simulink model "VoltageSourceConverterHVDCTrans"  (R2025b)
settings: Solver=FixedStepDiscrete  StartTime=0.0  StopTime=5  FixedStep=Ts  MaxStep=1e-4  RelTol=1e-3
PreLoadFcn:
  | VoltageSourceConverterHVDCTransParameters
values from neighbouring files (symbols this model uses):
  c = 0.207e-6    (= 2.07e-07)    [VoltageSourceConverterHVDCTransParameters.m]
  Cf = ((QRatedFilter/(VRated^2*(2*pi*FRated)))*(n^2-1)/(n^2))/Cbase    [VoltageSourceConverterHVDCTransParameters.m]
  FRated = 60    [VoltageSourceConverterHVDCTransParameters.m]
  Idcbase = Pbase/VdcRated    (= 1000)    [VoltageSourceConverterHVDCTransParameters.m]
  IL0 = opIdc.get("I").Value.value    [VoltageSourceConverterHVDCTransInitializeModel.m]
  l = 0.189e-3    (= 0.000189)    [VoltageSourceConverterHVDCTransParameters.m]
  Lbase = Zbase/wbase    [VoltageSourceConverterHVDCTransParameters.m]
  Lr = 0.15    [VoltageSourceConverterHVDCTransParameters.m]
  n = 25    [VoltageSourceConverterHVDCTransParameters.m]
  PRated = 300e6    (= 300000000)    [VoltageSourceConverterHVDCTransParameters.m]
  r = 0.0376    [VoltageSourceConverterHVDCTransParameters.m]
  Rc = r*Dis    (= 11.28)    [VoltageSourceConverterHVDCTransParameters.m]
  Rr = 0.002    [VoltageSourceConverterHVDCTransParameters.m]
  Rt = 0.002625    [VoltageSourceConverterHVDCTransParameters.m]
  Ts = 1/(fsw*100)    [VoltageSourceConverterHVDCTransInitializeModel.m]    (also in VoltageSourceConverterHVDCTransParameters.m = 6.66666666667e-05; VoltageSourceConverterHVDCTransVariantControl.m)
  Tsc = 10*Ts    (= 0.166666666667)    [VoltageSourceConverterHVDCTransInitializeModel.m]    (also in VoltageSourceConverterHVDCTransParameters.m = 6.66666666667e-05; VoltageSourceConverterHVDCTransVariantControl.m)
  Vdcr0 = 2*opReceivingEndVdcp.get("V").Value.value    [VoltageSourceConverterHVDCTransInitializeModel.m]
  VdcRated = 300e3    (= 300000)    [VoltageSourceConverterHVDCTransParameters.m]
  Vdcs0 = 2*opSendingEndVdcp.get("V").Value.value    [VoltageSourceConverterHVDCTransInitializeModel.m]
  VRated = 150e3    (= 150000)    [VoltageSourceConverterHVDCTransParameters.m]
  Xt = 0.19197    [VoltageSourceConverterHVDCTransParameters.m]
  Zbase = Vbase/Ibase    [VoltageSourceConverterHVDCTransParameters.m]
undefined symbols (not defined in the file or in its folder): DiscIntNeverNeededParam
libraries: nesl_utility x43, fl_lib x32, ee_lib x22, eeTransforms x16, eeGeneralControl x14, slpidlib x13, mcbeeMathTransformLib x8, eeSinusoidalMeasurement x2, eePwmGeneratorThreeLevel x2
(part 2 of 4)

== system VoltageSourceConverterHVDCTrans/Sending end DC filter ==
  Bus Creator : BusCreator  Inputs=4
  Cfns : fl_lib/Electrical/Electrical Elements/Capacitor  c=Cdcf F  r=0 Ohm  g=0 1/Ohm  i_specify=off  i_priority=High  i=0 A  i_nominal_specify=off  i_nominal_value=1  i_nominal_unit=A  v_specify=off  v_priority=High  v=Vdcs0/2 V  v_nominal_specify=off  v_nominal_value=1  v_nominal_unit=V  vc_specify=on  vc_priority=High  vc=Vdcs0/2 V  vc_nominal_specify=off  vc_nominal_value=1  vc_nominal_unit=V
  Cfps : fl_lib/Electrical/Electrical Elements/Capacitor  c=Cdcf F  r=0 Ohm  g=0 1/Ohm  i_specify=off  i_priority=High  i=0 A  i_nominal_specify=off  i_nominal_value=1  i_nominal_unit=A  v_specify=off  v_priority=High  v=Vdcs0/2 V  v_nominal_specify=off  v_nominal_value=1  v_nominal_unit=V  vc_specify=on  vc_priority=High  vc=Vdcs0/2 V  vc_nominal_specify=off  vc_nominal_value=1  vc_nominal_unit=V
  Cns : fl_lib/Electrical/Electrical Elements/Capacitor  c=Cdc F  r=1e-3 Ohm  g=0 1/Ohm  i_specify=off  i_priority=High  i=0 A  i_nominal_specify=off  i_nominal_value=1  i_nominal_unit=A  v_specify=off  v_priority=High  v=Vdcs0/2 V  v_nominal_specify=off  v_nominal_value=1  v_nominal_unit=V  vc_specify=on  vc_priority=High  vc=Vdcs0/2 V  vc_nominal_specify=off  vc_nominal_value=1  vc_nominal_unit=V
  Cps : fl_lib/Electrical/Electrical Elements/Capacitor  c=Cdc F  r=1e-3 Ohm  g=0 1/Ohm  i_specify=off  i_priority=High  i=0 A  i_nominal_specify=off  i_nominal_value=1  i_nominal_unit=A  v_specify=off  v_priority=High  v=Vdcs0/2 V  v_nominal_specify=off  v_nominal_value=1  v_nominal_unit=V  vc_specify=on  vc_priority=High  vc=Vdcs0/2 V  vc_nominal_specify=off  vc_nominal_value=1  vc_nominal_unit=V
  Electrical Reference : fl_lib/Electrical/Electrical Elements/Electrical Reference
  Lfns : fl_lib/Electrical/Electrical Elements/Inductor  l=L2 H  r=0.05 Ohm  g=0 1/Ohm  i_specify=off  i_priority=None  i=0 A  i_nominal_specify=off  i_nominal_value=1  i_nominal_unit=A  v_specify=off  v_priority=None  v=0 V  v_nominal_specify=off  v_nominal_value=1  v_nominal_unit=V  i_L_specify=on  i_L_priority=High  i_L=-IL0 A  i_L_nominal_specify=off  i_L_nominal_value=1  i_L_nominal_unit=A
  Lfps : fl_lib/Electrical/Electrical Elements/Inductor  l=L2 H  r=0.05 Ohm  g=0 1/Ohm  i_specify=off  i_priority=High  i=0 A  i_nominal_specify=off  i_nominal_value=1  i_nominal_unit=A  v_specify=off  v_priority=None  v=0 V  v_nominal_specify=off  v_nominal_value=1  v_nominal_unit=V  i_L_specify=on  i_L_priority=High  i_L=IL0 A  i_L_nominal_specify=off  i_L_nominal_value=1  i_L_nominal_unit=A
  Lfs : fl_lib/Electrical/Electrical Elements/Inductor  l=L1 H  r=0.1 Ohm  g=0 1/Ohm  i_specify=off  i_priority=None  i=0 A  i_nominal_specify=off  i_nominal_value=1  i_nominal_unit=A  v_specify=off  v_priority=None  v=0 V  v_nominal_specify=off  v_nominal_value=1  v_nominal_unit=V  i_L_specify=on  i_L_priority=None  i_L=0 A  i_L_nominal_specify=off  i_L_nominal_value=1  i_L_nominal_unit=A
  Sensing current1 : Subsystem
      settings: PortSchema="{\"entries\":[{\"content\":{\"sides\":[{\"content\":{\"connectorIds\":[\"LConn1\"]},\"type\":\"ConnectorPlacement.EquallySpacedRectSide\",\"uuid\":\"b182dbc5-c8d5-4832-a7cd-ea3787954646\"},{\"content\":{\"connectorIds\":[\"RConn1\",\"Out1\"],\"side\":\"RIGHT\"},\"type\":\"ConnectorPlacement.EquallySpacedRectSide\",\"uuid\":\"bfc6f163-1abf-440b-aa89-1443f971fd07\"},{\"content\":{\"connectorIds\":[],\"side\":\"TOP\"},\"type\":\"ConnectorPlacement.EquallySpacedRectSide\",\"uuid\":\"dd2a104c-9a72-483e-91c4-dbef9b359450\"}]},\"type\":\"ConnectorPlacement.EquallySpacedConnector\",\"uuid\":\"ce98cc3b-f524-409d-a465-fff2e3b7df79\"}],\"packageUris\":[\"http://schema.mathworks.com/mf0/Connector/R2020b\"],\"version\":\"1.0\"}"
  Sensing current2 : Subsystem
      settings: PortSchema="{\"entries\":[{\"content\":{\"sides\":[{\"content\":{\"connectorIds\":[\"LConn1\"]},\"type\":\"ConnectorPlacement.EquallySpacedRectSide\",\"uuid\":\"b182dbc5-c8d5-4832-a7cd-ea3787954646\"},{\"content\":{\"connectorIds\":[\"RConn1\",\"Out1\"],\"side\":\"RIGHT\"},\"type\":\"ConnectorPlacement.EquallySpacedRectSide\",\"uuid\":\"bfc6f163-1abf-440b-aa89-1443f971fd07\"},{\"content\":{\"connectorIds\":[],\"side\":\"TOP\"},\"type\":\"ConnectorPlacement.EquallySpacedRectSide\",\"uuid\":\"dd2a104c-9a72-483e-91c4-dbef9b359450\"}]},\"type\":\"ConnectorPlacement.EquallySpacedConnector\",\"uuid\":\"ce98cc3b-f524-409d-a465-fff2e3b7df79\"}],\"packageUris\":[\"http://schema.mathworks.com/mf0/Connector/R2020b\"],\"version\":\"1.0\"}"
  Vdcn : Subsystem
      settings: PortSchema="{\"entries\":[{\"content\":{\"sides\":[{\"content\":{\"connectorIds\":[\"LConn1\",\"Out1\"]},\"type\":\"ConnectorPlacement.EquallySpacedRectSide\",\"uuid\":\"bc3757cc-4537-444e-89af-7b7d8c8c1fa7\"},{\"content\":{\"connectorIds\":[\"RConn1\"],\"side\":\"RIGHT\"},\"type\":\"ConnectorPlacement.EquallySpacedRectSide\",\"uuid\":\"908bf4c4-26f6-4d8a-bcf8-68236027f5f8\"},{\"content\":{\"side\":\"TOP\"},\"type\":\"ConnectorPlacement.EquallySpacedRectSide\",\"uuid\":\"33f228db-ba47-4718-96dc-a72de309ae8c\"},{\"content\":{\"side\":\"BOTTOM\"},\"type\":\"ConnectorPlacement.EquallySpacedRectSide\",\"uuid\":\"d9b66c7e-0954-4c47-8bcc-77bf13ff573c\"}]},\"type\":\"ConnectorPlacement.EquallySpacedConnector\",\"uuid\":\"345f3578-0572-4e64-b2f3-84728129a12d\"}],\"packageUris\":[\"http://schema.mathworks.com/mf0/Connector/R2020b\"],\"version\":\"1.0\"}"
  Vdcp : Subsystem
      settings: PortSchema="{\"entries\":[{\"content\":{\"sides\":[{\"content\":{\"connectorIds\":[\"LConn1\",\"Out1\"]},\"type\":\"ConnectorPlacement.EquallySpacedRectSide\",\"uuid\":\"bc3757cc-4537-444e-89af-7b7d8c8c1fa7\"},{\"content\":{\"connectorIds\":[\"RConn1\"],\"side\":\"RIGHT\"},\"type\":\"ConnectorPlacement.EquallySpacedRectSide\",\"uuid\":\"908bf4c4-26f6-4d8a-bcf8-68236027f5f8\"},{\"content\":{\"side\":\"TOP\"},\"type\":\"ConnectorPlacement.EquallySpacedRectSide\",\"uuid\":\"33f228db-ba47-4718-96dc-a72de309ae8c\"},{\"content\":{\"side\":\"BOTTOM\"},\"type\":\"ConnectorPlacement.EquallySpacedRectSide\",\"uuid\":\"d9b66c7e-0954-4c47-8bcc-77bf13ff573c\"}]},\"type\":\"ConnectorPlacement.EquallySpacedConnector\",\"uuid\":\"345f3578-0572-4e64-b2f3-84728129a12d\"}],\"packageUris\":[\"http://schema.mathworks.com/mf0/Connector/R2020b\"],\"version\":\"1.0\"}"
  +in : PMIOPort  Side=Left
  0 : PMIOPort  Port=2  Side=Left
  -in : PMIOPort  Port=3  Side=Left
  +out : PMIOPort  Port=4  Side=Right
  -out : PMIOPort  Port=5  Side=Right
  mDC : Outport
  wires:
  Vdcp/1(v) -> Bus Creator/1  "VdcpS"
  Vdcn/1(v) -> Bus Creator/2  "VdcnS"
  Sensing current1/1(i) -> Bus Creator/3  "IdcpS"
  Sensing current2/1(i) -> Bus Creator/4  "IdcnS"
  Bus Creator/1 -> mDC/1
  connections:
  0/RConn1 -- Vdcn/LConn1 -- Electrical Reference/LConn1 -- Cns/LConn1 -- Cps/RConn1 -- Lfs/LConn1 -- Vdcp/RConn1
  Cfps/LConn1 -- +in/RConn1 -- Vdcp/LConn1 -- Cps/LConn1 -- Lfps/LConn1
  Cfps/RConn1 -- Cfns/LConn1 -- Lfs/RConn1
  Lfns/LConn1 -- Cns/RConn1 -- Vdcn/RConn1 -- -in/RConn1 -- Cfns/RConn1
  Sensing current1/RConn1 -- +out/RConn1
  Lfps/RConn1 -- Sensing current1/LConn1
  Sensing current2/RConn1 -- -out/RConn1
  Lfns/RConn1 -- Sensing current2/LConn1

== system VoltageSourceConverterHVDCTrans/Sending end vi1 ==
  Current and Voltage Sensor (Three-Phase) : ee_lib/Sensors & Transducers/Current and Voltage Sensor (Three-Phase)  vMeasurementType=ee.enum.vmeasurement.lg  outputUnit=ee.enum.unit.pu  SRated=300 MW  VRated=150 kV  I_specify=off  I_priority=None  I=[0, 0, 0] A  I_nominal_specify=off  I_nominal_value=1  I_nominal_unit=A  V_specify=off  V_priority=None  V=[0, 0, 0] V  V_nominal_specify=off  V_nominal_value=1  V_nominal_unit=V
      settings: InternalSimscapePortConfiguration="{\"Bottom\":[],\"Left\":[{\"id\":\"N1\",\"label\":\"~1\",\"type\":\"foundation.electrical.three_phase\"}],\"Right\":[{\"id\":\"V_output\",\"label\":\"V\",\"type\":\"output\"},{\"id\":\"I_output\",\"label\":\"I\",\"type\":\"output\"},{\"id\":\"N2\",\"label\":\"~2\",\"type\":\"foundation.electrical.three_phase\"}],\"Top\":[]}"
  PS-Simulink Converter : nesl_utility/PS-Simulink Converter  PhysicalDomain=network_engine_domain  SubClassName=ps_output  LeftPortType=input  RightPortType=output  PseudoPeriodic=off  Frequencies=[]  VectorFormat=1-D array  Unit=1  AffineConversion=off
  PS-Simulink Converter2 : nesl_utility/PS-Simulink Converter  PhysicalDomain=network_engine_domain  SubClassName=ps_output  LeftPortType=input  RightPortType=output  PseudoPeriodic=off  Frequencies=[]  VectorFormat=1-D array  Unit=1  AffineConversion=off
  ~1 : PMIOPort  Side=Left
  ~2 : PMIOPort  Port=2  Side=Right
  v : Outport
  i : Outport  Port=2
  wires:
  PS-Simulink Converter/1 -> i/1
  PS-Simulink Converter2/1 -> v/1
  connections:
  Current and Voltage Sensor (Three-Phase)/LConn1 -- ~1/RConn1
  Current and Voltage Sensor (Three-Phase)/RConn2 -- PS-Simulink Converter/LConn1
  PS-Simulink Converter2/LConn1 -- Current and Voltage Sensor (Three-Phase)/RConn1
  ~2/RConn1 -- Current and Voltage Sensor (Three-Phase)/RConn3

== system VoltageSourceConverterHVDCTrans/Sending end vi2 ==
  Current and Voltage Sensor (Three-Phase) : ee_lib/Sensors & Transducers/Current and Voltage Sensor (Three-Phase)  vMeasurementType=ee.enum.vmeasurement.lg  outputUnit=ee.enum.unit.pu  SRated=300 MW  VRated=345 kV  I_specify=off  I_priority=None  I=[0, 0, 0] A  I_nominal_specify=off  I_nominal_value=1  I_nominal_unit=A  V_specify=off  V_priority=None  V=[0, 0, 0] V  V_nominal_specify=off  V_nominal_value=1  V_nominal_unit=V
      settings: InternalSimscapePortConfiguration="{\"Bottom\":[],\"Left\":[{\"id\":\"N1\",\"label\":\"~1\",\"type\":\"foundation.electrical.three_phase\"}],\"Right\":[{\"id\":\"V_output\",\"label\":\"V\",\"type\":\"output\"},{\"id\":\"I_output\",\"label\":\"I\",\"type\":\"output\"},{\"id\":\"N2\",\"label\":\"~2\",\"type\":\"foundation.electrical.three_phase\"}],\"Top\":[]}"
  PS-Simulink Converter : nesl_utility/PS-Simulink Converter  PhysicalDomain=network_engine_domain  SubClassName=ps_output  LeftPortType=input  RightPortType=output  PseudoPeriodic=off  Frequencies=[]  VectorFormat=1-D array  Unit=1  AffineConversion=off
  PS-Simulink Converter2 : nesl_utility/PS-Simulink Converter  PhysicalDomain=network_engine_domain  SubClassName=ps_output  LeftPortType=input  RightPortType=output  PseudoPeriodic=off  Frequencies=[]  VectorFormat=1-D array  Unit=1  AffineConversion=off
  ~1 : PMIOPort  Side=Left
  ~2 : PMIOPort  Port=2  Side=Right
  v : Outport
  i : Outport  Port=2
  wires:
  PS-Simulink Converter2/1 -> v/1
  PS-Simulink Converter/1 -> i/1
  connections:
  PS-Simulink Converter2/LConn1 -- Current and Voltage Sensor (Three-Phase)/RConn1
  Current and Voltage Sensor (Three-Phase)/RConn2 -- PS-Simulink Converter/LConn1
  Current and Voltage Sensor (Three-Phase)/LConn1 -- ~1/RConn1
  ~2/RConn1 -- Current and Voltage Sensor (Three-Phase)/RConn3

== system VoltageSourceConverterHVDCTrans/Control/Sending end and receiving end control ==
  PrefS : Inport
  QrefS : Inport  Port=2
  VabcgS : Inport  Port=3
  IabcgS : Inport  Port=4
  IabcrS : Inport  Port=5
  VdcpS : Inport  Port=6
  VdcnS : Inport  Port=7
  VdcRef : Inport  Port=8
  QrefR : Inport  Port=9
  VabcgR : Inport  Port=10
  IabcgR : Inport  Port=11
  IabcrR : Inport  Port=12
  VdcpR : Inport  Port=13
  VdcnR : Inport  Port=14
  Receiving end control : Subsystem  Variant=on  EmptyChoice=on
  Sending end control : Subsystem  Variant=on  EmptyChoice=on
  Ss : Outport
  mSEndCon : Outport  Port=2
  Sr : Outport  Port=3
  mREndCon : Outport  Port=4
  wires:
  QrefR/1 -> Receiving end control/2(Qref)
  VabcgR/1 -> Receiving end control/3(Vabcg)
  VdcnR/1 -> Receiving end control/7(Vdcn)
  VdcpR/1 -> Receiving end control/6(Vdcp)
  VdcnS/1 -> Sending end control/7(Vdcn)
  PrefS/1 -> Sending end control/1(Pref)
  IabcrR/1 -> Receiving end control/5(Iabcr)
  VdcRef/1 -> Receiving end control/1(VdcRef)
  Receiving end control/1(S) -> Sr/1
  Receiving end control/2(mREndCon) -> mREndCon/1
  IabcgR/1 -> Receiving end control/4(Iabcg)
  QrefS/1 -> Sending end control/2(Qref)
  IabcgS/1 -> Sending end control/4(Iabcg)
  VdcpS/1 -> Sending end control/6(Vdcp)
  VabcgS/1 -> Sending end control/3(Vabcg)
  IabcrS/1 -> Sending end control/5(Iabcr)
  Sending end control/1(S) -> Ss/1
  Sending end control/2(mSEndCon) -> mSEndCon/1

== system VoltageSourceConverterHVDCTrans/Receiving end Converter/Average-value VSC ==
  S : Inport
  Average-value VSC : ee_lib/Semiconductors & Converters/Converters/Average-Value Voltage Source Converter (Three-Phase)  port_option=ee.enum.threePhasePort.composite  frequency_option=ee.enum.converters.frequency.constant  input_option=ee.enum.converters.inputOption.ModWave  FRated=60 Hz  losses_parameterization=ee.enum.converters.losses.fixed  Pfixed=1 W  ks=0.01  kc1=1.7 V  kc2=0.01 Ohm  Ploss_vect=[100, 800, 1870, 3250, 4900] W  Irms_vect=[10, 100, 200, 300, 400] A  Vdc_nom=300 V  thermal_mass=30000 J/K  temperature_specify=off  temperature_priority=High  temperature=298.15 K  temperature_nominal_specify=off  temperature_nominal_value=1  temperature_nominal_unit=K
      settings: InternalSimscapePortConfiguration="{\"Bottom\":[],\"Left\":[{\"id\":\"ModWave\",\"label\":\"ModWave\",\"type\":\"input\"},{\"id\":\"N\",\"label\":\"~\",\"type\":\"foundation.electrical.three_phase\"}],\"Right\":[{\"id\":\"p\",\"label\":\"+\",\"type\":\"foundation.electrical.electrical\"},{\"id\":\"n\",\"label\":\"-\",\"type\":\"foundation.electrical.electrical\"}],\"Top\":[]}"
  Electrical Reference1 : fl_lib/Electrical/Electrical Elements/Electrical Reference
  Simulink-PS Converter : nesl_utility/Simulink-PS Converter  PhysicalDomain=network_engine_domain  SubClassName=ps_input  LeftPortType=input  RightPortType=output  PseudoPeriodic=off  Frequencies=[]  NoiseDistribution=none  NoiseParameters=[]  Unit=1  AffineConversion=off  FilteringAndDerivatives=provide  SimscapeFilterOrder=1  InputFilterTimeConstant=0.001  UdotUserProvided=0
  + : PMIOPort  Side=Right
  0 : PMIOPort  Port=2  Side=Right
  - : PMIOPort  Port=3  Side=Right
  ~ : PMIOPort  Port=4  Side=Left
  wires:
  S/1 -> Simulink-PS Converter/1
  connections:
  Electrical Reference1/LConn1 -- 0/RConn1
  Average-value VSC/RConn2 -- -/RConn1
  Average-value VSC/RConn1 -- +/RConn1
  Simulink-PS Converter/RConn1 -- Average-value VSC/LConn1
  ~/RConn1 -- Average-value VSC/LConn2

== system VoltageSourceConverterHVDCTrans/Receiving end Converter/Switching VSC ==
  S : Inport
  Gate : Subsystem
  Three-Level Converter (Three-Phase) : ee_lib/Semiconductors & Converters/Converters/Three-Level Converter (Three-Phase)  port_option=ee.enum.threePhasePort.composite  device_type=ee.enum.converters.switchingdevicethreelevel.igbt  Vf=0.8 V  Ron=0.001 Ohm  Rds=0.001 Ohm  Goff=1e-5 1/Ohm  Vth=0.5 V  Vgt=1 V  Vgt_off=-1 V  Ih=1 A  K=0  diode_param=ee.enum.converters.diode.nodynamics  diode_Vf=0.8 V  diode_Ron=0.001 Ohm  diode_Goff=1e-5 1/Ohm  diode_C=50 nF  diode_iRM=-235 A  diode_iF=300 A  diode_idot=-50 A/us  diode_trr_param=ee.enum.converters.diodetrr.trr_factor  diode_trr_factor=3  diode_trr=15 us  diode_Qrr=1500 s*uA  snubber_type=ee.enum.converters.snubber.exclude  Cs=1e-7 F  Rs=0.1 Ohm
      settings: InternalSimscapePortConfiguration="{\"Bottom\":[],\"Left\":[{\"id\":\"G\",\"label\":\"G\",\"type\":\"foundation.electrical.twenty_four_phase\"},{\"id\":\"N\",\"label\":\"~\",\"type\":\"foundation.electrical.three_phase\"}],\"Right\":[{\"id\":\"p\",\"label\":\"+\",\"type\":\"foundation.electrical.electrical\"},{\"id\":\"z\",\"label\":\"0\",\"type\":\"foundation.electrical.electrical\"},{\"id\":\"n\",\"label\":\"-\",\"type\":\"foundation.electrical.electrical\"}],\"Top\":[]}"
  + : PMIOPort  Side=Right
  0 : PMIOPort  Port=2  Side=Right
  - : PMIOPort  Port=3  Side=Right
  ~ : PMIOPort  Port=4  Side=Left
  wires:
  S/1 -> Gate/1(S)
  connections:
  Three-Level Converter (Three-Phase)/RConn3 -- -/RConn1
  Gate/RConn1 -- Three-Level Converter (Three-Phase)/LConn1
  Three-Level Converter (Three-Phase)/RConn2 -- 0/RConn1
  Three-Level Converter (Three-Phase)/RConn1 -- +/RConn1
  Three-Level Converter (Three-Phase)/LConn2 -- ~/RConn1

== system VoltageSourceConverterHVDCTrans/Receiving end DC filter/Sensing current1 ==
  Current Sensor : fl_lib/Electrical/Electrical Sensors/Current Sensor
  PS-Simulink Converter : nesl_utility/PS-Simulink Converter  PhysicalDomain=network_engine_domain  SubClassName=ps_output  LeftPortType=input  RightPortType=output  PseudoPeriodic=off  Frequencies=[]  VectorFormat=1-D array  Unit=A  AffineConversion=off
  + : PMIOPort  Side=Left
  - : PMIOPort  Port=2  Side=Right
  i : Outport
  wires:
  PS-Simulink Converter/1 -> i/1
  connections:
  PS-Simulink Converter/LConn1 -- Current Sensor/RConn1
  Current Sensor/LConn1 -- +/RConn1
  -/RConn1 -- Current Sensor/RConn2

== system VoltageSourceConverterHVDCTrans/Receiving end DC filter/Sensing current2 ==
  Current Sensor : fl_lib/Electrical/Electrical Sensors/Current Sensor
  PS-Simulink Converter : nesl_utility/PS-Simulink Converter  PhysicalDomain=network_engine_domain  SubClassName=ps_output  LeftPortType=input  RightPortType=output  PseudoPeriodic=off  Frequencies=[]  VectorFormat=1-D array  Unit=A  AffineConversion=off
  + : PMIOPort  Side=Left
  - : PMIOPort  Port=2  Side=Right
  i : Outport
  wires:
  PS-Simulink Converter/1 -> i/1
  connections:
  -/RConn1 -- Current Sensor/RConn2
  Current Sensor/LConn1 -- +/RConn1
  PS-Simulink Converter/LConn1 -- Current Sensor/RConn1

== system VoltageSourceConverterHVDCTrans/Receiving end DC filter/Vdcn ==
  PS-Simulink Converter : nesl_utility/PS-Simulink Converter  PhysicalDomain=network_engine_domain  SubClassName=ps_output  LeftPortType=input  RightPortType=output  PseudoPeriodic=off  Frequencies=[]  VectorFormat=1-D array  Unit=V  AffineConversion=off
  Voltage Sensor : fl_lib/Electrical/Electrical Sensors/Voltage Sensor
  + : PMIOPort  Side=Left
  - : PMIOPort  Port=2  Side=Right
  v : Outport
  wires:
  PS-Simulink Converter/1 -> v/1
  connections:
  PS-Simulink Converter/LConn1 -- Voltage Sensor/RConn1
  Voltage Sensor/RConn2 -- -/RConn1
  Voltage Sensor/LConn1 -- +/RConn1

== system VoltageSourceConverterHVDCTrans/Receiving end DC filter/Vdcp ==
  PS-Simulink Converter : nesl_utility/PS-Simulink Converter  PhysicalDomain=network_engine_domain  SubClassName=ps_output  LeftPortType=input  RightPortType=output  PseudoPeriodic=off  Frequencies=[]  VectorFormat=1-D array  Unit=V  AffineConversion=off
  Voltage Sensor : fl_lib/Electrical/Electrical Sensors/Voltage Sensor
  + : PMIOPort  Side=Left
  - : PMIOPort  Port=2  Side=Right
  v : Outport
  wires:
  PS-Simulink Converter/1 -> v/1
  connections:
  Voltage Sensor/LConn1 -- +/RConn1
  Voltage Sensor/RConn2 -- -/RConn1
  PS-Simulink Converter/LConn1 -- Voltage Sensor/RConn1

== system VoltageSourceConverterHVDCTrans/Sending end Converter/Average-value VSC ==
  S : Inport
  Average-value VSC : ee_lib/Semiconductors & Converters/Converters/Average-Value Voltage Source Converter (Three-Phase)  port_option=ee.enum.threePhasePort.composite  frequency_option=ee.enum.converters.frequency.constant  input_option=ee.enum.converters.inputOption.ModWave  FRated=60 Hz  losses_parameterization=ee.enum.converters.losses.fixed  Pfixed=1 W  ks=0.01  kc1=1.7 V  kc2=0.01 Ohm  Ploss_vect=[100, 800, 1870, 3250, 4900] W  Irms_vect=[10, 100, 200, 300, 400] A  Vdc_nom=300 V  thermal_mass=30000 J/K  temperature_specify=off  temperature_priority=High  temperature=298.15 K  temperature_nominal_specify=off  temperature_nominal_value=1  temperature_nominal_unit=K
      settings: InternalSimscapePortConfiguration="{\"Bottom\":[],\"Left\":[{\"id\":\"ModWave\",\"label\":\"ModWave\",\"type\":\"input\"},{\"id\":\"N\",\"label\":\"~\",\"type\":\"foundation.electrical.three_phase\"}],\"Right\":[{\"id\":\"p\",\"label\":\"+\",\"type\":\"foundation.electrical.electrical\"},{\"id\":\"n\",\"label\":\"-\",\"type\":\"foundation.electrical.electrical\"}],\"Top\":[]}"
  Electrical Reference1 : fl_lib/Electrical/Electrical Elements/Electrical Reference
  Simulink-PS Converter : nesl_utility/Simulink-PS Converter  PhysicalDomain=network_engine_domain  SubClassName=ps_input  LeftPortType=input  RightPortType=output  PseudoPeriodic=off  Frequencies=[]  NoiseDistribution=none  NoiseParameters=[]  Unit=1  AffineConversion=off  FilteringAndDerivatives=provide  SimscapeFilterOrder=1  InputFilterTimeConstant=0.001  UdotUserProvided=0
  + : PMIOPort  Side=Right
  0 : PMIOPort  Port=2  Side=Right
  - : PMIOPort  Port=3  Side=Right
  ~ : PMIOPort  Port=4  Side=Left
  wires:
  S/1 -> Simulink-PS Converter/1
  connections:
  ~/RConn1 -- Average-value VSC/LConn2
  Simulink-PS Converter/RConn1 -- Average-value VSC/LConn1
  Average-value VSC/RConn1 -- +/RConn1
  Average-value VSC/RConn2 -- -/RConn1
  Electrical Reference1/LConn1 -- 0/RConn1

== system VoltageSourceConverterHVDCTrans/Sending end Converter/Switching VSC ==
  S : Inport
  Gate : Subsystem
  Three-Level Converter (Three-Phase) : ee_lib/Semiconductors & Converters/Converters/Three-Level Converter (Three-Phase)  port_option=ee.enum.threePhasePort.composite  device_type=ee.enum.converters.switchingdevicethreelevel.igbt  Vf=0.8 V  Ron=0.001 Ohm  Rds=0.001 Ohm  Goff=1e-5 1/Ohm  Vth=0.5 V  Vgt=1 V  Vgt_off=-1 V  Ih=1 A  K=0  diode_param=ee.enum.converters.diode.nodynamics  diode_Vf=0.8 V  diode_Ron=0.001 Ohm  diode_Goff=1e-5 1/Ohm  diode_C=50 nF  diode_iRM=-235 A  diode_iF=300 A  diode_idot=-50 A/us  diode_trr_param=ee.enum.converters.diodetrr.trr_factor  diode_trr_factor=3  diode_trr=15 us  diode_Qrr=1500 s*uA  snubber_type=ee.enum.converters.snubber.exclude  Cs=1e-7 F  Rs=0.1 Ohm
      settings: InternalSimscapePortConfiguration="{\"Bottom\":[],\"Left\":[{\"id\":\"G\",\"label\":\"G\",\"type\":\"foundation.electrical.twenty_four_phase\"},{\"id\":\"N\",\"label\":\"~\",\"type\":\"foundation.electrical.three_phase\"}],\"Right\":[{\"id\":\"p\",\"label\":\"+\",\"type\":\"foundation.electrical.electrical\"},{\"id\":\"z\",\"label\":\"0\",\"type\":\"foundation.electrical.electrical\"},{\"id\":\"n\",\"label\":\"-\",\"type\":\"foundation.electrical.electrical\"}],\"Top\":[]}"
  + : PMIOPort  Side=Right
  0 : PMIOPort  Port=2  Side=Right
  - : PMIOPort  Port=3  Side=Right
  ~ : PMIOPort  Port=4  Side=Left
  wires:
  S/1 -> Gate/1(S)
  connections:
  Three-Level Converter (Three-Phase)/LConn2 -- ~/RConn1
  Three-Level Converter (Three-Phase)/RConn1 -- +/RConn1
  Three-Level Converter (Three-Phase)/RConn2 -- 0/RConn1
  Gate/RConn1 -- Three-Level Converter (Three-Phase)/LConn1
  Three-Level Converter (Three-Phase)/RConn3 -- -/RConn1

== system VoltageSourceConverterHVDCTrans/Sending end DC filter/Sensing current1 ==
  Current Sensor : fl_lib/Electrical/Electrical Sensors/Current Sensor
  PS-Simulink Converter : nesl_utility/PS-Simulink Converter  PhysicalDomain=network_engine_domain  SubClassName=ps_output  LeftPortType=input  RightPortType=output  PseudoPeriodic=off  Frequencies=[]  VectorFormat=1-D array  Unit=A  AffineConversion=off
  + : PMIOPort  Side=Left
  - : PMIOPort  Port=2  Side=Right
  i : Outport
  wires:
  PS-Simulink Converter/1 -> i/1
  connections:
  -/RConn1 -- Current Sensor/RConn2
  Current Sensor/LConn1 -- +/RConn1
  PS-Simulink Converter/LConn1 -- Current Sensor/RConn1

== system VoltageSourceConverterHVDCTrans/Sending end DC filter/Sensing current2 ==
  Current Sensor : fl_lib/Electrical/Electrical Sensors/Current Sensor
  PS-Simulink Converter : nesl_utility/PS-Simulink Converter  PhysicalDomain=network_engine_domain  SubClassName=ps_output  LeftPortType=input  RightPortType=output  PseudoPeriodic=off  Frequencies=[]  VectorFormat=1-D array  Unit=A  AffineConversion=off
  + : PMIOPort  Side=Left
  - : PMIOPort  Port=2  Side=Right
  i : Outport
  wires:
  PS-Simulink Converter/1 -> i/1
  connections:
  PS-Simulink Converter/LConn1 -- Current Sensor/RConn1
  Current Sensor/LConn1 -- +/RConn1
  -/RConn1 -- Current Sensor/RConn2

== system VoltageSourceConverterHVDCTrans/Sending end DC filter/Vdcn ==
  PS-Simulink Converter : nesl_utility/PS-Simulink Converter  PhysicalDomain=network_engine_domain  SubClassName=ps_output  LeftPortType=input  RightPortType=output  PseudoPeriodic=off  Frequencies=[]  VectorFormat=1-D array  Unit=V  AffineConversion=off
  Voltage Sensor : fl_lib/Electrical/Electrical Sensors/Voltage Sensor
  + : PMIOPort  Side=Left
  - : PMIOPort  Port=2  Side=Right
  v : Outport
  wires:
  PS-Simulink Converter/1 -> v/1
  connections:
  Voltage Sensor/LConn1 -- +/RConn1
  Voltage Sensor/RConn2 -- -/RConn1
  PS-Simulink Converter/LConn1 -- Voltage Sensor/RConn1

== system VoltageSourceConverterHVDCTrans/Sending end DC filter/Vdcp ==
  PS-Simulink Converter : nesl_utility/PS-Simulink Converter  PhysicalDomain=network_engine_domain  SubClassName=ps_output  LeftPortType=input  RightPortType=output  PseudoPeriodic=off  Frequencies=[]  VectorFormat=1-D array  Unit=V  AffineConversion=off
  Voltage Sensor : fl_lib/Electrical/Electrical Sensors/Voltage Sensor
  + : PMIOPort  Side=Left
  - : PMIOPort  Port=2  Side=Right
  v : Outport
  wires:
  PS-Simulink Converter/1 -> v/1
  connections:
  PS-Simulink Converter/LConn1 -- Voltage Sensor/RConn1
  Voltage Sensor/RConn2 -- -/RConn1
  Voltage Sensor/LConn1 -- +/RConn1

== system VoltageSourceConverterHVDCTrans/Control/Sending end and receiving end control/Receiving end control ==
  VdcRef : Inport
  Qref : Inport  Port=2
  Vabcg : Inport  Port=3
  Iabcg : Inport  Port=4
  Iabcr : Inport  Port=5
  Vdcp : Inport  Port=6
  Vdcn : Inport  Port=7
  Frequency-and-time mode : Subsystem  VariantControl=ControllerFrequencyAndTimeMode
  Time mode : Subsystem  VariantControl=ControllerTimeMode
  S : Outport
  mREndCon : Outport  Port=2

== system VoltageSourceConverterHVDCTrans/Control/Sending end and receiving end control/Sending end control ==
  Pref : Inport
  Qref : Inport  Port=2
  Vabcg : Inport  Port=3
  Iabcg : Inport  Port=4
  Iabcr : Inport  Port=5
  Vdcp : Inport  Port=6
  Vdcn : Inport  Port=7
  Frequency-and-time mode : Subsystem  VariantControl=ControllerFrequencyAndTimeMode
  Time mode : Subsystem  VariantControl=ControllerTimeMode
  S : Outport
  mSEndCon : Outport  Port=2

== system VoltageSourceConverterHVDCTrans/Receiving end Converter/Switching VSC/Gate ==
  S : Inport
  Demux : Demux  Outputs=12
  Simulink-PS Converter{1..12} (12 alike) : nesl_utility/Simulink-PS Converter  PhysicalDomain=network_engine_domain  SubClassName=ps_input  LeftPortType=input  RightPortType=output  PseudoPeriodic=off  Frequencies=[]  NoiseDistribution=none  NoiseParameters=[]  Unit=1  AffineConversion=off  FilteringAndDerivatives=zero  SimscapeFilterOrder=1  InputFilterTimeConstant=0.001  UdotUserProvided=1
  Twelve-Pulse Gate Multiplexer : ee_lib/Semiconductors & Converters/Converters/Twelve-Pulse Gate Multiplexer  port_option=ee.enum.controlport.ps
      settings: InternalSimscapePortConfiguration="{\"Bottom\":[],\"Left\":[{\"id\":\"Ga1_ps\",\"label\":\"Ga(1)\",\"type\":\"input\"},{\"id\":\"Ga2_ps\",\"label\":\"Ga(2)\",\"type\":\"input\"},{\"id\":\"Ga3_ps\",\"label\":\"Ga(3)\",\"type\":\"input\"},{\"id\":\"Ga4_ps\",\"label\":\"Ga(4)\",\"type\":\"input\"},{\"id\":\"Gb1_ps\",\"label\":\"Gb(1)\",\"type\":\"input\"},{\"id\":\"Gb2_ps\",\"label\":\"Gb(2)\",\"type\":\"input\"},{\"id\":\"Gb3_ps\",\"label\":\"Gb(3)\",\"type\":\"input\"},{\"id\":\"Gb4_ps\",\"label\":\"Gb(4)\",\"type\":\"input\"},{\"id\":\"Gc1_ps\",\"label\":\"Gc(1)\",\"type\":\"input\"},{\"id\":\"Gc2_ps\",\"label\":\"Gc(2)\",\"type\":\"input\"},{\"id\":\"Gc3_ps\",\"label\":\"Gc(3)\",\"type\":\"input\"},{\"id\":\"Gc4_ps\",\"label\":\"Gc(4)\",\"type\":\"input\"}],\"Right\":[{\"id\":\"p\",\"label\":\"G\",\"type\":\"foundation.electrical.twenty_four_phase\"}],\"Top\":[]}"
  G : PMIOPort  Side=Right
  wires:
  Demux/9 -> Simulink-PS Converter9/1
  Demux/12 -> Simulink-PS Converter12/1
  Demux/11 -> Simulink-PS Converter11/1
  Demux/8 -> Simulink-PS Converter8/1
  Demux/7 -> Simulink-PS Converter7/1
  Demux/10 -> Simulink-PS Converter10/1
  Demux/4 -> Simulink-PS Converter4/1
  Demux/1 -> Simulink-PS Converter1/1
  Demux/2 -> Simulink-PS Converter2/1
  S/1 -> Demux/1
  Demux/5 -> Simulink-PS Converter5/1
  Demux/6 -> Simulink-PS Converter6/1
  Demux/3 -> Simulink-PS Converter3/1
  connections:
  Twelve-Pulse Gate Multiplexer/LConn7 -- Simulink-PS Converter7/RConn1
  Twelve-Pulse Gate Multiplexer/LConn11 -- Simulink-PS Converter11/RConn1
  Twelve-Pulse Gate Multiplexer/LConn12 -- Simulink-PS Converter12/RConn1
  Twelve-Pulse Gate Multiplexer/LConn9 -- Simulink-PS Converter9/RConn1
  Twelve-Pulse Gate Multiplexer/LConn8 -- Simulink-PS Converter8/RConn1
  Twelve-Pulse Gate Multiplexer/LConn10 -- Simulink-PS Converter10/RConn1
  Twelve-Pulse Gate Multiplexer/LConn4 -- Simulink-PS Converter4/RConn1
  Twelve-Pulse Gate Multiplexer/LConn2 -- Simulink-PS Converter2/RConn1
  Twelve-Pulse Gate Multiplexer/LConn3 -- Simulink-PS Converter3/RConn1
  Twelve-Pulse Gate Multiplexer/LConn6 -- Simulink-PS Converter6/RConn1
  Twelve-Pulse Gate Multiplexer/LConn5 -- Simulink-PS Converter5/RConn1
  Twelve-Pulse Gate Multiplexer/LConn1 -- Simulink-PS Converter1/RConn1
  Twelve-Pulse Gate Multiplexer/RConn1 -- G/RConn1

== system VoltageSourceConverterHVDCTrans/Sending end Converter/Switching VSC/Gate ==
  S : Inport
  Demux : Demux  Outputs=12
  Simulink-PS Converter{1..12} (12 alike) : nesl_utility/Simulink-PS Converter  PhysicalDomain=network_engine_domain  SubClassName=ps_input  LeftPortType=input  RightPortType=output  PseudoPeriodic=off  Frequencies=[]  NoiseDistribution=none  NoiseParameters=[]  Unit=1  AffineConversion=off  FilteringAndDerivatives=zero  SimscapeFilterOrder=1  InputFilterTimeConstant=0.001  UdotUserProvided=1
  Twelve-Pulse Gate Multiplexer : ee_lib/Semiconductors & Converters/Converters/Twelve-Pulse Gate Multiplexer  port_option=ee.enum.controlport.ps
      settings: InternalSimscapePortConfiguration="{\"Bottom\":[],\"Left\":[{\"id\":\"Ga1_ps\",\"label\":\"Ga(1)\",\"type\":\"input\"},{\"id\":\"Ga2_ps\",\"label\":\"Ga(2)\",\"type\":\"input\"},{\"id\":\"Ga3_ps\",\"label\":\"Ga(3)\",\"type\":\"input\"},{\"id\":\"Ga4_ps\",\"label\":\"Ga(4)\",\"type\":\"input\"},{\"id\":\"Gb1_ps\",\"label\":\"Gb(1)\",\"type\":\"input\"},{\"id\":\"Gb2_ps\",\"label\":\"Gb(2)\",\"type\":\"input\"},{\"id\":\"Gb3_ps\",\"label\":\"Gb(3)\",\"type\":\"input\"},{\"id\":\"Gb4_ps\",\"label\":\"Gb(4)\",\"type\":\"input\"},{\"id\":\"Gc1_ps\",\"label\":\"Gc(1)\",\"type\":\"input\"},{\"id\":\"Gc2_ps\",\"label\":\"Gc(2)\",\"type\":\"input\"},{\"id\":\"Gc3_ps\",\"label\":\"Gc(3)\",\"type\":\"input\"},{\"id\":\"Gc4_ps\",\"label\":\"Gc(4)\",\"type\":\"input\"}],\"Right\":[{\"id\":\"p\",\"label\":\"G\",\"type\":\"foundation.electrical.twenty_four_phase\"}],\"Top\":[]}"
  G : PMIOPort  Side=Right
  wires:
  Demux/3 -> Simulink-PS Converter3/1
  Demux/6 -> Simulink-PS Converter6/1
  Demux/5 -> Simulink-PS Converter5/1
  S/1 -> Demux/1
  Demux/2 -> Simulink-PS Converter2/1
  Demux/1 -> Simulink-PS Converter1/1
  Demux/4 -> Simulink-PS Converter4/1
  Demux/10 -> Simulink-PS Converter10/1
  Demux/7 -> Simulink-PS Converter7/1
  Demux/8 -> Simulink-PS Converter8/1
  Demux/11 -> Simulink-PS Converter11/1
  Demux/12 -> Simulink-PS Converter12/1
  Demux/9 -> Simulink-PS Converter9/1
  connections:
  Twelve-Pulse Gate Multiplexer/RConn1 -- G/RConn1
  Twelve-Pulse Gate Multiplexer/LConn1 -- Simulink-PS Converter1/RConn1
  Twelve-Pulse Gate Multiplexer/LConn5 -- Simulink-PS Converter5/RConn1
  Twelve-Pulse Gate Multiplexer/LConn6 -- Simulink-PS Converter6/RConn1
  Twelve-Pulse Gate Multiplexer/LConn3 -- Simulink-PS Converter3/RConn1
  Twelve-Pulse Gate Multiplexer/LConn2 -- Simulink-PS Converter2/RConn1
  Twelve-Pulse Gate Multiplexer/LConn4 -- Simulink-PS Converter4/RConn1
  Twelve-Pulse Gate Multiplexer/LConn10 -- Simulink-PS Converter10/RConn1
  Twelve-Pulse Gate Multiplexer/LConn8 -- Simulink-PS Converter8/RConn1
  Twelve-Pulse Gate Multiplexer/LConn9 -- Simulink-PS Converter9/RConn1
  Twelve-Pulse Gate Multiplexer/LConn12 -- Simulink-PS Converter12/RConn1
  Twelve-Pulse Gate Multiplexer/LConn11 -- Simulink-PS Converter11/RConn1
  Twelve-Pulse Gate Multiplexer/LConn7 -- Simulink-PS Converter7/RConn1

== system VoltageSourceConverterHVDCTrans/Control/Sending end and receiving end control/Receiving end control/Frequency-and-time mode ==
  VdcRef : Inport
  Qref : Inport  Port=2
  Vabcg : Inport  Port=3
  Iabcg : Inport  Port=4
  Iabcr : Inport  Port=5
  Vdcp : Inport  Port=6
  Vdcn : Inport  Port=7
  Bus Creator : BusCreator  Inputs=4
  Control : Subsystem
  Measurements : Subsystem
  S : Outport
  mREndCon : Outport  Port=2
  wires:
  VdcRef/1 -> Bus Creator/1, Control/1(VdcRef)  "VdcRef"
  Qref/1 -> Bus Creator/2, Control/2(Qref)  "Qref"
  Iabcg/1 -> Measurements/2(Iabcg)
  Iabcr/1 -> Measurements/3(Iabcr)
  Vabcg/1 -> Measurements/1(Vabcg)
  Vdcp/1 -> Measurements/4(Vdcp)
  Control/1(S) -> S/1
  Vdcn/1 -> Measurements/5(Vdcn)
  Measurements/1(omega) -> Control/3(omega)
  Measurements/2(theta) -> Control/4(theta)
  Measurements/3(Vdg) -> Control/5(Vd)
  Measurements/4(idr) -> Control/6(idr)
  Measurements/5(iqr) -> Control/7(iqr)
  Measurements/6(VdcpF) -> Control/8(Vdcp)
  Measurements/7(VdcnF) -> Control/9(Vdcn)
  Measurements/8(Qmea) -> Bus Creator/3, Control/10(Qmea)  "Qmea"
  Bus Creator/1 -> mREndCon/1
  Measurements/9(Pmea) -> Bus Creator/4  "Pmea"

== system VoltageSourceConverterHVDCTrans/Control/Sending end and receiving end control/Receiving end control/Time mode ==
  VdcRef : Inport
  Qref : Inport  Port=2
  Vabcg : Inport  Port=3
  Iabcg : Inport  Port=4
  Iabcr : Inport  Port=5
  Vdcp : Inport  Port=6
  Vdcn : Inport  Port=7
  Bus Creator : BusCreator  Inputs=4
  Measurements : Subsystem
  Receiving-end Control : Subsystem
  S : Outport
  mREndCon : Outport  Port=2
  wires:
  Receiving-end Control/1(S) -> S/1
  Vdcn/1 -> Measurements/5(Vdcn)
  Vdcp/1 -> Measurements/4(Vdcp)
  Iabcr/1 -> Measurements/3(Iabcr)
  Iabcg/1 -> Measurements/2(Iabcg)
  Vabcg/1 -> Measurements/1(Vabcg)
  Qref/1 -> Bus Creator/2, Receiving-end Control/2(Qref)  "Qref"
  Measurements/1(omega) -> Receiving-end Control/3(omega)
  Measurements/2(theta) -> Receiving-end Control/4(theta)
  Measurements/3(Vdg) -> Receiving-end Control/5(Vd)
  Measurements/4(idg) -> Receiving-end Control/6(idg)
  Measurements/5(iqg) -> Receiving-end Control/7(iqg)
  Measurements/6(idr) -> Receiving-end Control/8(idr)
  Measurements/7(iqr) -> Receiving-end Control/9(iqr)
  Measurements/8(VdcpF) -> Receiving-end Control/10(Vdcp)
  Measurements/9(VdcnF) -> Receiving-end Control/11(Vdcn)
  Measurements/10(Qmea) -> Bus Creator/3, Receiving-end Control/12(Qmea)  "Qmea"
  VdcRef/1 -> Bus Creator/1, Receiving-end Control/1(VdcRef)  "VdcRef"
  Bus Creator/1 -> mREndCon/1
  Measurements/11(Pmea) -> Bus Creator/4  "Pmea"

== system VoltageSourceConverterHVDCTrans/Control/Sending end and receiving end control/Sending end control/Frequency-and-time mode ==
  Pref : Inport
  Qref : Inport  Port=2
  Vabcg : Inport  Port=3
  Iabcg : Inport  Port=4
  Iabcr : Inport  Port=5
  Vdcp : Inport  Port=6
  Vdcn : Inport  Port=7
  Bus Creator : BusCreator  Inputs=4
  Control : Subsystem
  Measurements : Subsystem
  S : Outport
  mSEndCon : Outport  Port=2
  wires:
  Vdcn/1 -> Measurements/5(Vdcn)
  Control/1(S) -> S/1
  Vdcp/1 -> Measurements/4(Vdcp)
  Vabcg/1 -> Measurements/1(Vabcg)
  Iabcr/1 -> Measurements/3(Iabcr)
  Iabcg/1 -> Measurements/2(Iabcg)
  Measurements/1(omega) -> Control/3(omega)
  Measurements/2(theta) -> Control/4(theta)
  Measurements/3(Vdg) -> Control/5(Vd)
  Measurements/4(idr) -> Control/6(idr)
  Measurements/5(iqr) -> Control/7(iqr)
  Measurements/6(VdcpF) -> Control/8(Vdcp)
  Measurements/7(VdcnF) -> Control/9(Vdcn)
  Measurements/8(Pmea) -> Bus Creator/3, Control/10(Pmea)  "Pmea"
  Measurements/9(Qmea) -> Bus Creator/4, Control/11(Qmea)  "Qmea"
  Qref/1 -> Bus Creator/2, Control/2(Qref)  "Qref"
  Pref/1 -> Bus Creator/1, Control/1(Pref)  "Pref"
  Bus Creator/1 -> mSEndCon/1

== system VoltageSourceConverterHVDCTrans/Control/Sending end and receiving end control/Sending end control/Time mode ==
  Pref : Inport
  Qref : Inport  Port=2
  Vabcg : Inport  Port=3
  Iabcg : Inport  Port=4
  Iabcr : Inport  Port=5
  Vdcp : Inport  Port=6
  Vdcn : Inport  Port=7
  Bus Creator : BusCreator  Inputs=4
  Control : Subsystem
  Measurements : Subsystem
  S : Outport
  mSEndCon : Outport  Port=2
  wires:
  Measurements/1(omega) -> Control/3(omega)
  Qref/1 -> Bus Creator/2, Control/2(Qref)  "Qref"
  Measurements/10(Pmea) -> Bus Creator/3, Control/12(Pmea)  "Pmea"
  Measurements/3(Vdg) -> Control/5(Vd)
  Measurements/8(VdcpF) -> Control/10(Vdcp)
  Measurements/7(iqr) -> Control/9(iqr)
  Measurements/9(VdcnF) -> Control/11(Vdcn)
  Measurements/6(idr) -> Control/8(idr)
  Measurements/11(Qmea) -> Bus Creator/4, Control/13(Qmea)  "Qmea"
  Measurements/4(idg) -> Control/6(idg)
  Measurements/5(iqg) -> Control/7(iqg)
  Pref/1 -> Bus Creator/1, Control/1(Pref)  "Pref"
  Measurements/2(theta) -> Control/4(theta)
  Vabcg/1 -> Measurements/1(Vabcg)
  Iabcg/1 -> Measurements/2(Iabcg)
  Iabcr/1 -> Measurements/3(Iabcr)
  Vdcp/1 -> Measurements/4(Vdcp)
  Vdcn/1 -> Measurements/5(Vdcn)
  Control/1(S) -> S/1
  Bus Creator/1 -> mSEndCon/1

== system VoltageSourceConverterHVDCTrans/Control/Sending end and receiving end control/Receiving end control/Frequency-and-time mode/Control ==
  VdcRef : Inport
  Qref : Inport  Port=2
  omega : Inport  Port=3
  theta : Inport  Port=4
  Vd : Inport  Port=5
  idr : Inport  Port=6
  iqr : Inport  Port=7
  Vdcp : Inport  Port=8
  Vdcn : Inport  Port=9
  Qmea : Inport  Port=10
  Current control : Subsystem
  DC voltage and reactive power control : Subsystem
  Unit Delay1 : UnitDelay  InitialCondition=Vdgr0  SampleTime=Tsc  HasFrameUpgradeWarning=on
  Unit Delay2 : UnitDelay  InitialCondition=1  SampleTime=Tsc  HasFrameUpgradeWarning=on
  Unit Delay3 : UnitDelay  InitialCondition=Vdcr0/2/(VdcRated/2)  SampleTime=Tsc  HasFrameUpgradeWarning=on
  Unit Delay4 : UnitDelay  InitialCondition=Vdcr0/2/(VdcRated/2)  SampleTime=Tsc  HasFrameUpgradeWarning=on
  Unit Delay5 : UnitDelay  InitialCondition=Idr0  SampleTime=Tsc  HasFrameUpgradeWarning=on
  Unit Delay6 : UnitDelay  InitialCondition=Iqr0  SampleTime=Tsc  HasFrameUpgradeWarning=on
  Unit Delay8 : UnitDelay  InitialCondition=Qr0  SampleTime=Tsc  HasFrameUpgradeWarning=on
  Unit Delay9 : UnitDelay  InitialCondition=-pi/6+Vphaser0  SampleTime=Tsc  HasFrameUpgradeWarning=on
  S : Outport
  wires:
  idr/1 -> Unit Delay5/1
  Unit Delay8/1 -> DC voltage and reactive power control/5(Qmea)
  DC voltage and reactive power control/1(idRef) -> Current control/1(idgRef)
  omega/1 -> Unit Delay2/1
  iqr/1 -> Unit Delay6/1
  Qref/1 -> DC voltage and reactive power control/4(Qref)
  Vdcn/1 -> Unit Delay4/1
  Unit Delay4/1 -> Current control/7(Vdcn), DC voltage and reactive power control/3(Vdcn)
  Unit Delay6/1 -> Current control/4(iqr)
  Unit Delay5/1 -> Current control/3(idr)
  DC voltage and reactive power control/2(iqRef) -> Current control/2(iqgRef)
  Vd/1 -> Unit Delay1/1
  theta/1 -> Unit Delay9/1
  Unit Delay1/1 -> Current control/5(Vd)
  Unit Delay3/1 -> Current control/6(Vdcp), DC voltage and reactive power control/2(Vdcp)
  Qmea/1 -> Unit Delay8/1
  VdcRef/1 -> DC voltage and reactive power control/1(VdcRef)
  Unit Delay2/1 -> Current control/8(omega)
  Vdcp/1 -> Unit Delay3/1
  Current control/1(S) -> S/1
  Unit Delay9/1 -> Current control/9(theta)

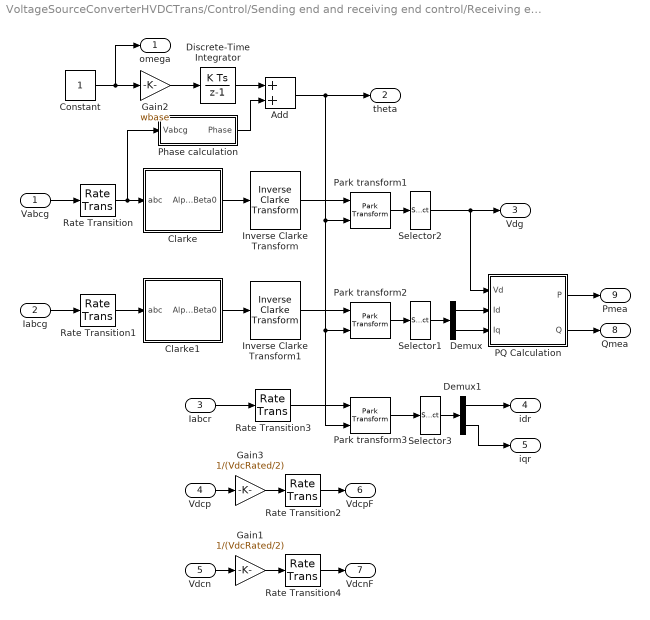
== system VoltageSourceConverterHVDCTrans/Control/Sending end and receiving end control/Receiving end control/Frequency-and-time mode/Measurements ==
  Vabcg : Inport
  Iabcg : Inport  Port=2
  Iabcr : Inport  Port=3
  Vdcp : Inport  Port=4
  Vdcn : Inport  Port=5
  Add : Sum
  Clarke : Subsystem
  Clarke1 : Subsystem
  Constant : Constant  SampleTime=Tsc
  Demux : Demux  Outputs=2
  Demux1 : Demux  Outputs=2
  Discrete-Time Integrator : DiscreteIntegrator  InitialCondition=-pi/6  SampleTime=Tsc  ICPrevOutput=DiscIntNeverNeededParam  ICPrevScaledInput=DiscIntNeverNeededParam
  Gain1 : Gain  Gain=1/(VdcRated/2)
  Gain2 : Gain  Gain=wbase
  Gain3 : Gain  Gain=1/(VdcRated/2)
  Inverse Clarke Transform : mcbeeMathTransformLib/Inverse Clarke Transform  PowerInvariant=off  UseWithEmbedded=off  PhaseInput=Two inputs
      settings: LibrarySourceBlock=|
      | ee_sl_lib/Mathematical
      | Transforms/Inverse
      | Clarke Transform
  Inverse Clarke Transform1 : mcbeeMathTransformLib/Inverse Clarke Transform  PowerInvariant=off  UseWithEmbedded=off  PhaseInput=Two inputs
      settings: LibrarySourceBlock=|
      | ee_sl_lib/Mathematical
      | Transforms/Inverse
      | Clarke Transform
  PQ Calculation : Subsystem
  Park transform1 : eeTransforms/Park Transform  AxisAlignment=Q-axis  PowerInvariant=off
  Park transform2 : eeTransforms/Park Transform  AxisAlignment=Q-axis  PowerInvariant=off
  Park transform3 : eeTransforms/Park Transform  AxisAlignment=Q-axis  PowerInvariant=off
  Phase calculation : Subsystem
  Rate Transition : RateTransition  InitialCondition=Vabcgr0  OutPortSampleTime=Tsc
  Rate Transition1 : RateTransition  InitialCondition=Iabcgr0  OutPortSampleTime=Tsc
  Rate Transition2 : RateTransition  InitialCondition=Vdcr0/2/(VdcRated/2)  OutPortSampleTime=Tsc
  Rate Transition3 : RateTransition  InitialCondition=Iabcrr0  OutPortSampleTime=Tsc
  Rate Transition4 : RateTransition  InitialCondition=Vdcr0/2/(VdcRated/2)  OutPortSampleTime=Tsc
  Selector1 : Selector  InputPortWidth=3  IndexOptions=Index vector (dialog)  Indices=[1 2]  OutputSizes=1
  Selector2 : Selector  InputPortWidth=3  IndexOptions=Index vector (dialog)  Indices=[1]  OutputSizes=1
  Selector3 : Selector  InputPortWidth=3  IndexOptions=Index vector (dialog)  Indices=[1 2]  OutputSizes=1
  omega : Outport  VectorParamsAs1DForOutWhenUnconnected=off
  theta : Outport  Port=2  VectorParamsAs1DForOutWhenUnconnected=off
  Vdg : Outport  Port=3  VectorParamsAs1DForOutWhenUnconnected=off
  idr : Outport  Port=4  VectorParamsAs1DForOutWhenUnconnected=off
  iqr : Outport  Port=5  VectorParamsAs1DForOutWhenUnconnected=off
  VdcpF : Outport  Port=6  VectorParamsAs1DForOutWhenUnconnected=off
  VdcnF : Outport  Port=7  VectorParamsAs1DForOutWhenUnconnected=off
  Qmea : Outport  Port=8  VectorParamsAs1DForOutWhenUnconnected=off
  Pmea : Outport  Port=9  VectorParamsAs1DForOutWhenUnconnected=off
  wires:
  Rate Transition3/1 -> Park transform3/1
  Gain2/1 -> Discrete-Time Integrator/1
  Demux/1 -> PQ Calculation/2(Id)
  Gain3/1 -> Rate Transition2/1
  Inverse Clarke Transform1/1 -> Park transform2/1
  Selector2/1 -> PQ Calculation/1(Vd), Vdg/1
  Constant/1 -> Gain2/1, omega/1
  Clarke1/1(AlphaBeta0) -> Inverse Clarke Transform1/1
  Iabcg/1 -> Rate Transition1/1
  Rate Transition2/1 -> VdcpF/1
  Gain1/1 -> Rate Transition4/1
  Park transform1/1 -> Selector2/1
  Demux1/2 -> iqr/1
  Demux1/1 -> idr/1
  Rate Transition/1 -> Phase calculation/1(Vabcg), Clarke/1(abc)
  Park transform2/1 -> Selector1/1
  Vdcn/1 -> Gain1/1
  Inverse Clarke Transform/1 -> Park transform1/1
  Iabcr/1 -> Rate Transition3/1
  Rate Transition4/1 -> VdcnF/1
  Vabcg/1 -> Rate Transition/1
  Demux/2 -> PQ Calculation/3(Iq)
  PQ Calculation/2(Q) -> Qmea/1
  Add/1 -> theta/1, Park transform1/2, Park transform2/2, Park transform3/2
  Vdcp/1 -> Gain3/1
  Selector1/1 -> Demux/1
  Clarke/1(AlphaBeta0) -> Inverse Clarke Transform/1
  PQ Calculation/1(P) -> Pmea/1
  Rate Transition1/1 -> Clarke1/1(abc)
  Selector3/1 -> Demux1/1
  Park transform3/1 -> Selector3/1
  Discrete-Time Integrator/1 -> Add/1
  Phase calculation/1(Phase) -> Add/2
